simulink model "jumeau_banc_rw"  (R2025b)
settings: Solver=ode23t  StartTime=0.0  StopTime=20  MaxStep=1e-3  RelTol=1e-4
PostLoadFcn:
  | d = fileparts(get_param('jumeau_banc_rw', 'FileName')); addpath(fullfile(d, 'geometrie'), fullfile(d, 'liaison'), fullfile(d, 'pilotage')); clear d
StartFcn:
  | % Jumeau Webots : au lancement, MATLAB envoie les paramètres du Model Workspace à Webots, qui remet le banc en
  | % position de départ, puis ouvre la liaison de télémétrie et la liaison de commande (liaison/pont_banc.m).
  | if strcmp(get_param('jumeau_banc_rw/Procédé', 'LabelModeActiveChoice'), 'Webots')
  |     pont_banc('ouvrir', getVariable(get_param('jumeau_banc_rw', 'ModelWorkspace'), 'config_jumeau'));
  | end
  | pilotage_banc('depart');   % interface de pilotage : nouveau lancement
StopFcn:
  | pont_banc('fermer');
  | pilotage_banc('fin');
model workspace (MATLAB code in the model file):
  | %% Jumeau numérique du banc de stabilisation à 4 roues de réaction (version 3) : paramètres
  | % Ce code est enregistré dans le modèle (Model Explorer > jumeau_banc_rw > Model Workspace).
  | % Origine : (CAO) CAO du banc version 3, (M) mesuré sur le matériel, (F) fiche technique, (Fw) firmware,
  | % (H) hypothèse à mesurer sur le banc. Masses et inerties des pièces : dans chaque bloc de pièce.
  | 
  | %% Montage de l'essai
  | pivot_mm = 25;              % position du pivot de tangage sur le corps : 25, 24, 16, 8, 0, -8 mm (25 : banc équilibré, rangée +24 et paliers remontés de 1 mm)
  | blocage_roulis = 0;         % goupille de blocage : 1 = axe bloqué à 0°, 0 = axe libre
  | blocage_tangage = 0;
  | angle0_roulis_deg = 2;      % position de départ (mise à 0 si l'axe est bloqué)
  | angle0_tangage_deg = -1;
  | g = 9.81;                   % m/s²
  | 
  | %% Pupitre : pilotage manuel des 4 ESC
  | essai_t = 1;                % s, instant de l'échelon d'essai ajouté aux curseurs
  | essai_echelon_us = [0 0 0 0];   % µs, échelon d'essai sur chaque ESC (0 : aucun)
  | 
  | %% Alimentation des ESC
  | V_alim = 12;                % V, alimentation de labo (H : tension réglée)
  | 
  | %% ESC Brushless 30A bidirectionnels (x4)
  | f_trame_esc = 50;           % Hz, une impulsion toutes les 20 ms (Fw : LEDC 50 Hz)
  | imp_neutre = 1500;          % µs, neutre (testé sur le banc)
  | imp_min = 1000;             % µs (Fw)
  | imp_max = 2000;             % µs (Fw)
  | zone_morte_us = 0;          % µs autour du neutre (H)
  | tau_esc = 2e-3;             % s, temps de réponse de l'ESC (H)
  | armement_actif = 1;         % 1 : l'ESC ne pilote le moteur qu'après t_armement au neutre
  | t_armement = 1;             % s (H)
  | fenetre_armement_us = 25;   % µs, écart au neutre accepté pendant l'armement (H)
  | sens_moteurs = [1 1 1 1];   % +1 : au-dessus du neutre, la roue tourne dans le sens +axe (vers l'extérieur) (H : ordre des phases)
  | 
  | %% Moteurs A2212 1400 KV (x4), modèle équivalent continu
  | KV = 1400;                  % tr/min/V (F)
  | Ke = 60/(2*pi*KV);          % V.s/rad
  | Kt = Ke;                    % N.m/A
  | R_moteur = 0.08;            % ohm (H)
  | L_moteur = 30e-6;           % H (H)
  | f_roue = 5e-6;              % N.m.s/rad, frottement visqueux des roulements du moteur (H)
  | 
  | %% Cardan
  | butee_deg = 20;             % débattement de chaque axe (CAO)
  | k_butee = 20;               % N.m/rad, contact goupille-lumière (H)
  | c_butee = 0.2;              % N.m.s/rad (H)
  | b_cardan = 1e-4;            % N.m.s/rad, frottement des roulements 625 (H)
  | k_cables = 0;               % N.m/rad, raideur des deux câbles vers la table (H)
  | 
  | %% BNO055 (mode fusion)
  | T_bno = 0.01;               % s, données de fusion à 100 Hz (F)
  | bruit_bno = 1;              % 1 : bruit de mesure, 0 : capteur parfait
  | sigma_angle_deg = 0.05;     % ° (H)
  | sigma_gyro_dps = 0.1;       % °/s (H)
  | sigma_acc = 0.02;           % m/s² (H)
  | R_montage_bno = eye(3);     % axes du capteur dans le repère du dispositif : eye(3) = remappage AXIS_MAP réglé
  |                             % (la carte est tournée de 90° dans la CAO)
  | 
  | %% Capteurs de vitesse TCRT5000 (x4) : un front à chaque rayon du disque
  | n_rayons = 4;               % rayons du disque vus par tour (CAO : disque d'origine)
  | T_tcrt = 1e-3;              % s, pas de calcul du capteur (les fronts sont datés par interpolation, comme un chronomètre en µs)
  | t_arret_tcrt = 0.2;         % s sans front : la vitesse mesurée retombe à 0 (Fw, à fixer)
  | 
  | %% Pont vers le jumeau Webots (et, plus tard, vers l'ESP32 du banc réel)
  | T_pont = 0.01;              % s, une trame de commande et une trame de télémétrie toutes les 10 ms
  | 
  | %% Essai : maintien au départ et perturbation
  | t_lacher = 2;                % s, le dispositif est tenu à la main à sa position de départ jusqu'à cet instant (0 : libre dès le départ)
  | k_main = 5;                  % N.m/rad, raideur de la main qui tient le dispositif
  | c_main = 0.3;                % N.m.s/rad, son amortissement
  | perturbation_t = 7;          % s, instant de la poussée d'essai
  | perturbation_duree = 0.2;    % s
  | perturbation_couple = [0.02 0.02];   % N.m, couple de la poussée sur [roulis tangage], programmée (0 : aucune ; l'interface de pilotage en ajoute)
  | 
  | %% Grandeurs dérivées
  | assert(any(pivot_mm == [25 24 16 8 0 -8]), 'pivot_mm : 25, 24, 16, 8, 0, -8');
  | q0_deg = [angle0_roulis_deg angle0_tangage_deg] .* ([blocage_roulis blocage_tangage] == 0);
  | config_jumeau = [pivot_mm; blocage_roulis; blocage_tangage; q0_deg(:); V_alim; f_trame_esc; imp_neutre; imp_min; imp_max; ...
  |     zone_morte_us; tau_esc; armement_actif; t_armement; fenetre_armement_us; sens_moteurs(:); Ke; Kt; R_moteur; L_moteur; ...
  |     f_roue; butee_deg; k_butee; c_butee; b_cardan; k_cables; g; T_bno; bruit_bno; sigma_angle_deg; sigma_gyro_dps; ...
  |     sigma_acc; n_rayons; t_arret_tcrt; T_tcrt; R_montage_bno(:); T_pont; t_lacher; k_main; c_main];   % 51 valeurs envoyées au jumeau Webots au lancement
  | 
  | %% Commande bas niveau : une boucle de vitesse par roue, avec observateur CFO (méthode du TP2, ramenée à la vitesse)
  | J_roue = 1.562e-4;          % kg.m², inertie d'une roue autour de son axe : disque, vis, cloche du moteur (CAO)
  | T_cbn = 1/f_trame_esc;      % s, période de calcul de la commande : celle des ESC, qui ne lisent qu'une impulsion toutes les 20 ms
  | wc_roue = [10 10 10 10];    % rad/s, rapidité du suivi de vitesse de chaque roue (pôle de l'erreur en -wc)
  | wo_roue = [5 5 5 5];        % rad/s, rapidité du CFO de chaque roue (pôles en -wo et -4 wo) ; au-delà de 10, il devient instable à 20 ms
  | imp_cmd_min = 1375;         % µs, limites des impulsions commandées : vitesse conseillée des disques, 3 900 tr/min
  | imp_cmd_max = 1625;         % µs
  | w_aveugle = 45;             % rad/s, en dessous (vitesse du modèle), le TCRT5000 voit mal la roue : le CFO ne se corrige plus sur la mesure
  | 
  | %% Consigne d'essai des roues : ajoutée à la consigne qui vient de la conversion (0 tant qu'elle est vide)
  | essai_roue_t1 = 2;                  % s, départ vers le premier palier
  | essai_roue_vitesse1 = [0 0 0 0];  % rad/s, premier palier de chaque roue (0 : la roue reste à l'arrêt)
  | essai_roue_t2 = 6;                  % s, départ vers le second palier
  | essai_roue_vitesse2 = [0 0 0 0];    % rad/s, second palier de chaque roue
  | essai_roue_acc = 300;               % rad/s², pente des rampes entre les paliers
  | 
  | %% Commande bas niveau : grandeurs calculées
  | % modèle local d'une roue : d(omega)/dt = -a1 omega + a0 V + d
  | a0_roue = Kt/(R_moteur*J_roue) * [1 1 1 1];                % rad/s² par volt
  | a1_roue = (Kt*Ke/R_moteur + f_roue)/J_roue * [1 1 1 1];    % 1/s
  | K_roue = wc_roue - a1_roue;                                % retour d'état : erreur en -(a1 + K) = -wc
  | l1_roue = 5*wo_roue;                                       % CFO
  | lambda_roue = 4/5*wo_roue;
  | 
  | %% Référence : angles demandés au dispositif, en polynômes de degré 5 entre deux paliers
  | ref_t = [2 12];              % s, instant de départ vers chaque palier
  | ref_roulis_deg = [0 5];      % °, roulis demandé à chaque palier
  | ref_tangage_deg = [0 0];     % °, tangage demandé à chaque palier
  | ref_duree = 1.5;             % s, durée du passage d'un palier au suivant
  | 
  | %% Commande haut niveau : une boucle par axe [roulis tangage], placement de pôles basé sur l'observateur CFO (TP2)
  | T_chn = T_cbn;               % s, période de calcul : celle de la commande bas niveau et des ESC
  | t_depart = t_lacher;         % s, mise en marche de la commande : au moment où la main lâche le dispositif
  | wc_axe = [4 4];              % rad/s, rapidité du suivi d'angle de chaque axe
  | xi_axe = [1 1];              % amortissement
  | wo_axe = [3 3];              % rad/s, rapidité du CFO de chaque axe (pôles en -wo et -4 wo, double) ; au-delà de 4, le couple s'agite
  | desat_active = 0;            % 1 : la référence est décalée pour ramener les roues vers leur vitesse de repos
  | T_desat = 5;                 % s, constante de temps de ce retour
  | desat_max_deg = 15;          % °, décalage maximal de la référence
  | 
  | %% Conversion : couples des deux axes vers les 4 roues
  | w_repos = 200;               % rad/s, vitesse de repos des 4 roues : elles tournent toujours, le TCRT5000 les voit toujours
  | t_roues = t_armement + 0.2;  % s, mise en rotation des roues, une fois les ESC armés
  | acc_roue_max = 300;          % rad/s², accélération maximale demandée à une roue
  | w_roue_min = 60;             % rad/s, vitesses limites demandées à une roue
  | w_roue_max = 400;            % rad/s (disques : 3 900 tr/min conseillés, soit 408 rad/s)
  | 
  | %% Masses et inerties utilisées par la commande (CAO du banc version 3)
  | m_disp = 1.2615;             % kg, dispositif et ses 4 roues
  | zG_disp = 24.977e-3;         % m, hauteur de son centre de masse sur le corps (le pivot est à pivot_mm)
  | Ixx_disp_24 = 8.2684e-3;     % kg.m², inertie du dispositif autour du roulis, pivot à +24 mm
  | Iyy_disp_24 = 8.2786e-3;     % kg.m², autour du tangage, pivot à +24 mm
  | m_croix = 0.0755;            % kg, croisillon et paliers (ne tournent qu'en roulis)
  | zG_croix = 0.257e-3;         % m, hauteur de leur centre de masse au-dessus de l'axe de roulis
  | Ixx_croix = 2.073e-4;        % kg.m²
  | 
  | %% Commande haut niveau et conversion : grandeurs calculées
  | % modèle local d'un axe : d²(theta)/dt² = -a1 d(theta)/dt + a0 C + d, avec C le couple demandé aux roues
  | hz = zG_disp - pivot_mm/1000;                                    % m, centre de masse du dispositif au-dessus du pivot
  | I_axe = [Ixx_disp_24 + Ixx_croix, Iyy_disp_24] + m_disp*(hz^2 - (zG_disp - 0.024)^2) - 2*J_roue;   % kg.m²
  | mgh_axe = g*[m_disp*hz + m_croix*zG_croix, m_disp*hz];           % N.m/rad, couple de pesanteur par radian d'inclinaison
  | a0_axe = 1./I_axe;                                               % rad/s² par N.m
  | a1_axe = b_cardan./I_axe;                                        % 1/s
  | k1_axe = wc_axe.^2;                                              % retour d'état : s² + 2 xi wc s + wc²
  | k2_axe = 2*xi_axe.*wc_axe - a1_axe;
  | l1_axe = 9*wo_axe;                                               % CFO du TP2
  | l2_axe = 12*wo_axe.^2;
  | lambda_axe = 4/3*wo_axe;
  | C_max = 2*J_roue*cosd(45)*acc_roue_max;                          % N.m, couple maximal demandé sur un axe
  | k_desat = desat_active.*sign(mgh_axe + (mgh_axe == 0))./(max(abs(mgh_axe), 1e-3)*T_desat);            % rad par N.m.s
  | sx_roues = [1 -1 -1 1];                                          % signe de cos(45°, 135°, 225°, 315°) : part de chaque roue sur le roulis
  | sy_roues = [1 1 -1 -1];                                          % signe de sin : part sur le tangage
  | M_conv = -[sx_roues(:) sy_roues(:)]/(4*J_roue*cosd(45));         % accélération des 4 roues pour un couple [roulis; tangage]
  | 
  | %% Perception : des mesures à l'état du banc
  | T_perception = T_bno;        % s, période de calcul : celle du BNO055
  | tau_desequilibre = 2;        % s, constante de temps du filtre du couple extérieur et du déséquilibre
  | 
  | %% Pilotage par l'interface (pilotage/pilote_banc.m)
  | manche_max_deg = 15;         % °, limite de sécurité de l'inclinaison demandée par le manche (l'interface règle l'amplitude)
  | w_manche = 3;                % rad/s, rapidité avec laquelle la référence rejoint le manche (second ordre critique)
  | T_affichage = 0.1;           % s, rafraîchissement de l'interface
undefined symbols (not defined in the file): DiscIntNeverNeededParam, X, Y, Z
libraries: sm_lib x256, nesl_utility x24, simulink x7
(part 3 of 8)

== system jumeau_banc_rw/Procédé/Jumeau Simscape/Mécanique (CAO version 3)/Croisillon (tourne en roulis) ==
  Collier 1 : sm_lib/Body Elements/File Solid  Description=|  ExtGeomFileName=RW-05_Collier.stl  UnitType=Custom  ExtGeomFileUnits=mm  StepReaderType=HEX  ExportConvexHullGeometry=off  InertiaType=Custom  BasedOnType=DensityFromFile  Density=1000  DensityUnits=kg/m^3  Mass=0.005537042  MassUnits=kg  CenterOfMass=[-0.00035108193 2.2209262e-05 0.0029842808]  CenterOfMassUnits=m  MomentsOfInertia=[3.8543243e-07 3.7829745e-07 7.2925271e-07]  MomentsOfInertiaUnits=kg*m^2  ProductsOfInertia=[-1.9330542e-12 3.0559842e-11 -4.3174034e-11]  ProductsOfInertiaUnits=kg*m^2  GraphicType=FromGeometry  MarkerShape=Sphere  MarkerSize=10  GraphicVisPropType=SimpleVisualProperties  GraphicDiffuseColor=[0.867 0.518 0.322]  GraphicOpacity=1  GraphicSpecularColor=[0.5 0.5 0.5 1.0]  GraphicAmbientColor=[0.15 0.15 0.15 1.0]  GraphicEmissiveColor=[0.0 0.0 0.0 1.0]  GraphicShininess=75  DoExposeReferenceFrame=on  SerializedFrames=<Frames/>
      | Pièce CAO : Collier 1 (RW-05_Collier)
      | Masse 5.54 g : PLA plein (hypothèse de conception), 1240 kg/m³.
      | Centre de masse et inertie : calculés sur la géométrie de la CAO.
  Collier 2 : sm_lib/Body Elements/File Solid  Description=|  ExtGeomFileName=RW-05_Collier.stl  UnitType=Custom  ExtGeomFileUnits=mm  StepReaderType=HEX  ExportConvexHullGeometry=off  InertiaType=Custom  BasedOnType=DensityFromFile  Density=1000  DensityUnits=kg/m^3  Mass=0.005537042  MassUnits=kg  CenterOfMass=[-0.00035108193 2.2209262e-05 0.0029842808]  CenterOfMassUnits=m  MomentsOfInertia=[3.8543243e-07 3.7829745e-07 7.2925271e-07]  MomentsOfInertiaUnits=kg*m^2  ProductsOfInertia=[-1.9330542e-12 3.0559842e-11 -4.3174034e-11]  ProductsOfInertiaUnits=kg*m^2  GraphicType=FromGeometry  MarkerShape=Sphere  MarkerSize=10  GraphicVisPropType=SimpleVisualProperties  GraphicDiffuseColor=[0.867 0.518 0.322]  GraphicOpacity=1  GraphicSpecularColor=[0.5 0.5 0.5 1.0]  GraphicAmbientColor=[0.15 0.15 0.15 1.0]  GraphicEmissiveColor=[0.0 0.0 0.0 1.0]  GraphicShininess=75  DoExposeReferenceFrame=on  SerializedFrames=<Frames/>
      | Pièce CAO : Collier 2 (RW-05_Collier)
      | Masse 5.54 g : PLA plein (hypothèse de conception), 1240 kg/m³.
      | Centre de masse et inertie : calculés sur la géométrie de la CAO.
  Croisillon : sm_lib/Body Elements/File Solid  Description=|  ExtGeomFileName=RW-06_Croisillon.stl  UnitType=Custom  ExtGeomFileUnits=mm  StepReaderType=HEX  ExportConvexHullGeometry=off  InertiaType=Custom  BasedOnType=DensityFromFile  Density=1000  DensityUnits=kg/m^3  Mass=0.025623078  MassUnits=kg  CenterOfMass=[-4.3032906e-14 1.5829923e-12 -4.8306735e-05]  CenterOfMassUnits=m  MomentsOfInertia=[3.4638965e-06 3.4316654e-06 3.4293676e-06]  MomentsOfInertiaUnits=kg*m^2  ProductsOfInertia=[-6.2250551e-17 3.045946e-18 -4.6836641e-17]  ProductsOfInertiaUnits=kg*m^2  GraphicType=FromGeometry  MarkerShape=Sphere  MarkerSize=10  GraphicVisPropType=SimpleVisualProperties  GraphicDiffuseColor=[0.91 0.639 0.239]  GraphicOpacity=1  GraphicSpecularColor=[0.5 0.5 0.5 1.0]  GraphicAmbientColor=[0.15 0.15 0.15 1.0]  GraphicEmissiveColor=[0.0 0.0 0.0 1.0]  GraphicShininess=75  DoExposeReferenceFrame=on  SerializedFrames=<Frames/>
      | Pièce CAO : Croisillon (RW-06_Croisillon)
      | Masse 25.62 g : PLA plein (hypothèse de conception), 1240 kg/m³.
      | Centre de masse et inertie : calculés sur la géométrie de la CAO.
  Entretoise de roulis 1 : sm_lib/Body Elements/File Solid  Description=|  ExtGeomFileName=RW-23_Entretoise-roulis-8x4.stl  UnitType=Custom  ExtGeomFileUnits=mm  StepReaderType=HEX  ExportConvexHullGeometry=off  InertiaType=Custom  BasedOnType=DensityFromFile  Density=1000  DensityUnits=kg/m^3  Mass=9.5479284e-05  MassUnits=kg  CenterOfMass=[-2.0837187e-19 -2.3504414e-20 0.002]  CenterOfMassUnits=m  MomentsOfInertia=[6.6443636e-10 6.6443636e-10 1.0742613e-09]  MomentsOfInertiaUnits=kg*m^2  ProductsOfInertia=[4.6214258e-28 1.1368684e-26 -3.8597625e-27]  ProductsOfInertiaUnits=kg*m^2  GraphicType=FromGeometry  MarkerShape=Sphere  MarkerSize=10  GraphicVisPropType=SimpleVisualProperties  GraphicDiffuseColor=[0.867 0.518 0.322]  GraphicOpacity=1  GraphicSpecularColor=[0.5 0.5 0.5 1.0]  GraphicAmbientColor=[0.15 0.15 0.15 1.0]  GraphicEmissiveColor=[0.0 0.0 0.0 1.0]  GraphicShininess=75  DoExposeReferenceFrame=on  SerializedFrames=<Frames/>
      | Pièce CAO : Entretoise de roulis 1 (RW-23_Entretoise-roulis-8x4)
      | Masse 0.10 g : PLA imprimé, 2 parois et 15 % de remplissage (hypothèse de conception), 800 kg/m³.
      | Centre de masse et inertie : calculés sur la géométrie de la CAO.
  Entretoise de roulis 2 : sm_lib/Body Elements/File Solid  Description=|  ExtGeomFileName=RW-23_Entretoise-roulis-8x4.stl  UnitType=Custom  ExtGeomFileUnits=mm  StepReaderType=HEX  ExportConvexHullGeometry=off  InertiaType=Custom  BasedOnType=DensityFromFile  Density=1000  DensityUnits=kg/m^3  Mass=9.5479284e-05  MassUnits=kg  CenterOfMass=[-2.0837187e-19 -2.3504414e-20 0.002]  CenterOfMassUnits=m  MomentsOfInertia=[6.6443636e-10 6.6443636e-10 1.0742613e-09]  MomentsOfInertiaUnits=kg*m^2  ProductsOfInertia=[4.6214258e-28 1.1368684e-26 -3.8597625e-27]  ProductsOfInertiaUnits=kg*m^2  GraphicType=FromGeometry  MarkerShape=Sphere  MarkerSize=10  GraphicVisPropType=SimpleVisualProperties  GraphicDiffuseColor=[0.867 0.518 0.322]  GraphicOpacity=1  GraphicSpecularColor=[0.5 0.5 0.5 1.0]  GraphicAmbientColor=[0.15 0.15 0.15 1.0]  GraphicEmissiveColor=[0.0 0.0 0.0 1.0]  GraphicShininess=75  DoExposeReferenceFrame=on  SerializedFrames=<Frames/>
      | Pièce CAO : Entretoise de roulis 2 (RW-23_Entretoise-roulis-8x4)
      | Masse 0.10 g : PLA imprimé, 2 parois et 15 % de remplissage (hypothèse de conception), 800 kg/m³.
      | Centre de masse et inertie : calculés sur la géométrie de la CAO.
  Goupille de butée de roulis : sm_lib/Body Elements/File Solid  Description=|  ExtGeomFileName=RW-24_Goupille-3x16.stl  UnitType=Custom  ExtGeomFileUnits=mm  StepReaderType=HEX  ExportConvexHullGeometry=off  InertiaType=Custom  BasedOnType=DensityFromFile  Density=1000  DensityUnits=kg/m^3  Mass=0.00088781408  MassUnits=kg  CenterOfMass=[-3.8480785e-19 5.0963439e-20 0.008]  CenterOfMassUnits=m  MomentsOfInertia=[1.9439429e-08 1.9439429e-08 9.9879084e-10]  MomentsOfInertiaUnits=kg*m^2  ProductsOfInertia=[2.3957297e-27 -4.1833204e-25 1.4074912e-26]  ProductsOfInertiaUnits=kg*m^2  GraphicType=FromGeometry  MarkerShape=Sphere  MarkerSize=10  GraphicVisPropType=SimpleVisualProperties  GraphicDiffuseColor=[0.314 0.314 0.314]  GraphicOpacity=1  GraphicSpecularColor=[0.5 0.5 0.5 1.0]  GraphicAmbientColor=[0.15 0.15 0.15 1.0]  GraphicEmissiveColor=[0.0 0.0 0.0 1.0]  GraphicShininess=75  DoExposeReferenceFrame=on  SerializedFrames=<Frames/>
      | Pièce CAO : Goupille de butée de roulis (RW-24_Goupille-3x16)
      | Masse 0.89 g : acier, 7850 kg/m³.
      | Centre de masse et inertie : calculés sur la géométrie de la CAO.
  Goupille de butée de tangage : sm_lib/Body Elements/File Solid  Description=|  ExtGeomFileName=RW-24_Goupille-3x16.stl  UnitType=Custom  ExtGeomFileUnits=mm  StepReaderType=HEX  ExportConvexHullGeometry=off  InertiaType=Custom  BasedOnType=DensityFromFile  Density=1000  DensityUnits=kg/m^3  Mass=0.00088781408  MassUnits=kg  CenterOfMass=[-3.8480785e-19 5.0963439e-20 0.008]  CenterOfMassUnits=m  MomentsOfInertia=[1.9439429e-08 1.9439429e-08 9.9879084e-10]  MomentsOfInertiaUnits=kg*m^2  ProductsOfInertia=[2.3957297e-27 -4.1833204e-25 1.4074912e-26]  ProductsOfInertiaUnits=kg*m^2  GraphicType=FromGeometry  MarkerShape=Sphere  MarkerSize=10  GraphicVisPropType=SimpleVisualProperties  GraphicDiffuseColor=[0.314 0.314 0.314]  GraphicOpacity=1  GraphicSpecularColor=[0.5 0.5 0.5 1.0]  GraphicAmbientColor=[0.15 0.15 0.15 1.0]  GraphicEmissiveColor=[0.0 0.0 0.0 1.0]  GraphicShininess=75  DoExposeReferenceFrame=on  SerializedFrames=<Frames/>
      | Pièce CAO : Goupille de butée de tangage (RW-24_Goupille-3x16)
      | Masse 0.89 g : acier, 7850 kg/m³.
      | Centre de masse et inertie : calculés sur la géométrie de la CAO.
  Pose Collier 1 : sm_lib/Frames and Transforms/Rigid Transform  RotationMethod=RotationMatrix  FollAlignAxisA=+X  BaseAlignAxisA=+Y  FollAlignAxisB=+Y  BaseAlignAxisB=+Z  RotationStandardAxis=+Z  RotationAngle=0  RotationAngleUnits=deg  RotationArbitraryAxis=[0 0 1]  RotationSequenceAxes=FollowerAxes  RotationSequence=XYX  RotationSequenceAngles=[0 0 0]  RotationSequenceAnglesUnits=deg  RotationMatrix=[-1 0 0;0 0 1;0 1 0]  Quaternion=[1 0 0 0]  TranslationMethod=Cartesian  TranslationCartesianOffset=[0 88.5 0]  TranslationCartesianOffsetUnits=mm  TranslationStandardAxis=+Z  TranslationStandardOffset=0  TranslationStandardOffsetUnits=m  TranslationROffset=0  TranslationROffsetUnits=m  TranslationThetaOffset=0  TranslationThetaOffsetUnits=deg  TranslationZOffset=0  TranslationZOffsetUnits=m
  Pose Collier 2 : sm_lib/Frames and Transforms/Rigid Transform  RotationMethod=RotationMatrix  FollAlignAxisA=+X  BaseAlignAxisA=+Y  FollAlignAxisB=+Y  BaseAlignAxisB=+Z  RotationStandardAxis=+Z  RotationAngle=0  RotationAngleUnits=deg  RotationArbitraryAxis=[0 0 1]  RotationSequenceAxes=FollowerAxes  RotationSequence=XYX  RotationSequenceAngles=[0 0 0]  RotationSequenceAnglesUnits=deg  RotationMatrix=[1 0 0;0 0 -1;0 1 0]  Quaternion=[1 0 0 0]  TranslationMethod=Cartesian  TranslationCartesianOffset=[0 -88.5 0]  TranslationCartesianOffsetUnits=mm  TranslationStandardAxis=+Z  TranslationStandardOffset=0  TranslationStandardOffsetUnits=m  TranslationROffset=0  TranslationROffsetUnits=m  TranslationThetaOffset=0  TranslationThetaOffsetUnits=deg  TranslationZOffset=0  TranslationZOffsetUnits=m
  Pose Entretoise de roulis 1 : sm_lib/Frames and Transforms/Rigid Transform  RotationMethod=RotationMatrix  FollAlignAxisA=+X  BaseAlignAxisA=+Y  FollAlignAxisB=+Y  BaseAlignAxisB=+Z  RotationStandardAxis=+Z  RotationAngle=0  RotationAngleUnits=deg  RotationArbitraryAxis=[0 0 1]  RotationSequenceAxes=FollowerAxes  RotationSequence=XYX  RotationSequenceAngles=[0 0 0]  RotationSequenceAnglesUnits=deg  RotationMatrix=[0 0 1;1 0 0;0 1 0]  Quaternion=[1 0 0 0]  TranslationMethod=Cartesian  TranslationCartesianOffset=[14 0 0]  TranslationCartesianOffsetUnits=mm  TranslationStandardAxis=+Z  TranslationStandardOffset=0  TranslationStandardOffsetUnits=m  TranslationROffset=0  TranslationROffsetUnits=m  TranslationThetaOffset=0  TranslationThetaOffsetUnits=deg  TranslationZOffset=0  TranslationZOffsetUnits=m
  Pose Entretoise de roulis 2 : sm_lib/Frames and Transforms/Rigid Transform  RotationMethod=RotationMatrix  FollAlignAxisA=+X  BaseAlignAxisA=+Y  FollAlignAxisB=+Y  BaseAlignAxisB=+Z  RotationStandardAxis=+Z  RotationAngle=0  RotationAngleUnits=deg  RotationArbitraryAxis=[0 0 1]  RotationSequenceAxes=FollowerAxes  RotationSequence=XYX  RotationSequenceAngles=[0 0 0]  RotationSequenceAnglesUnits=deg  RotationMatrix=[0 0 -1;1 0 0;0 -1 0]  Quaternion=[1 0 0 0]  TranslationMethod=Cartesian  TranslationCartesianOffset=[-14 0 0]  TranslationCartesianOffsetUnits=mm  TranslationStandardAxis=+Z  TranslationStandardOffset=0  TranslationStandardOffsetUnits=m  TranslationROffset=0  TranslationROffsetUnits=m  TranslationThetaOffset=0  TranslationThetaOffsetUnits=deg  TranslationZOffset=0  TranslationZOffsetUnits=m
  Pose Goupille de butée de roulis : sm_lib/Frames and Transforms/Rigid Transform  RotationMethod=RotationMatrix  FollAlignAxisA=+X  BaseAlignAxisA=+Y  FollAlignAxisB=+Y  BaseAlignAxisB=+Z  RotationStandardAxis=+Z  RotationAngle=0  RotationAngleUnits=deg  RotationArbitraryAxis=[0 0 1]  RotationSequenceAxes=FollowerAxes  RotationSequence=XYX  RotationSequenceAngles=[0 0 0]  RotationSequenceAnglesUnits=deg  RotationMatrix=[0 0 1;1 0 0;0 1 0]  Quaternion=[1 0 0 0]  TranslationMethod=Cartesian  TranslationCartesianOffset=[8 0 11.5]  TranslationCartesianOffsetUnits=mm  TranslationStandardAxis=+Z  TranslationStandardOffset=0  TranslationStandardOffsetUnits=m  TranslationROffset=0  TranslationROffsetUnits=m  TranslationThetaOffset=0  TranslationThetaOffsetUnits=deg  TranslationZOffset=0  TranslationZOffsetUnits=m
  Pose Goupille de butée de tangage : sm_lib/Frames and Transforms/Rigid Transform  RotationMethod=RotationMatrix  FollAlignAxisA=+X  BaseAlignAxisA=+Y  FollAlignAxisB=+Y  BaseAlignAxisB=+Z  RotationStandardAxis=+Z  RotationAngle=0  RotationAngleUnits=deg  RotationArbitraryAxis=[0 0 1]  RotationSequenceAxes=FollowerAxes  RotationSequence=XYX  RotationSequenceAngles=[0 0 0]  RotationSequenceAnglesUnits=deg  RotationMatrix=[1 0 0;0 0 1;0 -1 0]  Quaternion=[1 0 0 0]  TranslationMethod=Cartesian  TranslationCartesianOffset=[0 82.5 11.5]  TranslationCartesianOffsetUnits=mm  TranslationStandardAxis=+Z  TranslationStandardOffset=0  TranslationStandardOffsetUnits=m  TranslationROffset=0  TranslationROffsetUnits=m  TranslationThetaOffset=0  TranslationThetaOffsetUnits=deg  TranslationZOffset=0  TranslationZOffsetUnits=m
  Pose Tige de tangage : sm_lib/Frames and Transforms/Rigid Transform  RotationMethod=RotationMatrix  FollAlignAxisA=+X  BaseAlignAxisA=+Y  FollAlignAxisB=+Y  BaseAlignAxisB=+Z  RotationStandardAxis=+Z  RotationAngle=0  RotationAngleUnits=deg  RotationArbitraryAxis=[0 0 1]  RotationSequenceAxes=FollowerAxes  RotationSequence=XYX  RotationSequenceAngles=[0 0 0]  RotationSequenceAnglesUnits=deg  RotationMatrix=[1 0 0;0 0 1;0 -1 0]  Quaternion=[1 0 0 0]  TranslationMethod=Cartesian  TranslationCartesianOffset=[0 0 0]  TranslationCartesianOffsetUnits=mm  TranslationStandardAxis=+Z  TranslationStandardOffset=0  TranslationStandardOffsetUnits=m  TranslationROffset=0  TranslationROffsetUnits=m  TranslationThetaOffset=0  TranslationThetaOffsetUnits=deg  TranslationZOffset=0  TranslationZOffsetUnits=m
  Pose Vis épaulée 1 : sm_lib/Frames and Transforms/Rigid Transform  RotationMethod=RotationMatrix  FollAlignAxisA=+X  BaseAlignAxisA=+Y  FollAlignAxisB=+Y  BaseAlignAxisB=+Z  RotationStandardAxis=+Z  RotationAngle=0  RotationAngleUnits=deg  RotationArbitraryAxis=[0 0 1]  RotationSequenceAxes=FollowerAxes  RotationSequence=XYX  RotationSequenceAngles=[0 0 0]  RotationSequenceAnglesUnits=deg  RotationMatrix=[0 0 -1;1 0 0;0 -1 0]  Quaternion=[1 0 0 0]  TranslationMethod=Cartesian  TranslationCartesianOffset=[23 0 0]  TranslationCartesianOffsetUnits=mm  TranslationStandardAxis=+Z  TranslationStandardOffset=0  TranslationStandardOffsetUnits=m  TranslationROffset=0  TranslationROffsetUnits=m  TranslationThetaOffset=0  TranslationThetaOffsetUnits=deg  TranslationZOffset=0  TranslationZOffsetUnits=m
  Pose Vis épaulée 2 : sm_lib/Frames and Transforms/Rigid Transform  RotationMethod=RotationMatrix  FollAlignAxisA=+X  BaseAlignAxisA=+Y  FollAlignAxisB=+Y  BaseAlignAxisB=+Z  RotationStandardAxis=+Z  RotationAngle=0  RotationAngleUnits=deg  RotationArbitraryAxis=[0 0 1]  RotationSequenceAxes=FollowerAxes  RotationSequence=XYX  RotationSequenceAngles=[0 0 0]  RotationSequenceAnglesUnits=deg  RotationMatrix=[0 0 1;1 0 0;0 1 0]  Quaternion=[1 0 0 0]  TranslationMethod=Cartesian  TranslationCartesianOffset=[-23 0 0]  TranslationCartesianOffsetUnits=mm  TranslationStandardAxis=+Z  TranslationStandardOffset=0  TranslationStandardOffsetUnits=m  TranslationROffset=0  TranslationROffsetUnits=m  TranslationThetaOffset=0  TranslationThetaOffsetUnits=deg  TranslationZOffset=0  TranslationZOffsetUnits=m
  Tige de tangage : sm_lib/Body Elements/File Solid  Description=|  ExtGeomFileName=RW-21_Tige-5x200.stl  UnitType=Custom  ExtGeomFileUnits=mm  StepReaderType=HEX  ExportConvexHullGeometry=off  InertiaType=Custom  BasedOnType=DensityFromFile  Density=1000  DensityUnits=kg/m^3  Mass=0.030826878  MassUnits=kg  CenterOfMass=[3.4740139e-19 -9.3482873e-20 0]  CenterOfMassUnits=m  MomentsOfInertia=[0.00010280443 0.00010280443 9.6333993e-08]  MomentsOfInertiaUnits=kg*m^2  ProductsOfInertia=[-8.2139303e-24 -1.1423253e-22 1.106194e-23]  ProductsOfInertiaUnits=kg*m^2  GraphicType=FromGeometry  MarkerShape=Sphere  MarkerSize=10  GraphicVisPropType=SimpleVisualProperties  GraphicDiffuseColor=[0.2 0.2 0.2]  GraphicOpacity=1  GraphicSpecularColor=[0.5 0.5 0.5 1.0]  GraphicAmbientColor=[0.15 0.15 0.15 1.0]  GraphicEmissiveColor=[0.0 0.0 0.0 1.0]  GraphicShininess=75  DoExposeReferenceFrame=on  SerializedFrames=<Frames/>
      | Pièce CAO : Tige de tangage (RW-21_Tige-5x200)
      | Masse 30.83 g : acier, 7850 kg/m³.
      | Centre de masse et inertie : calculés sur la géométrie de la CAO.
  Vis épaulée 1 : sm_lib/Body Elements/File Solid  Description=|  ExtGeomFileName=RW-22_Vis-epaulee-5x10-M4.stl  UnitType=Custom  ExtGeomFileUnits=mm  StepReaderType=HEX  ExportConvexHullGeometry=off  InertiaType=Custom  BasedOnType=DensityFromFile  Density=1000  DensityUnits=kg/m^3  Mass=0.003  MassUnits=kg  CenterOfMass=[-4.1357308e-19 -6.3568799e-20 0.0032357143]  CenterOfMassUnits=m  MomentsOfInertia=[1.0565385e-07 1.0565385e-07 1.7426786e-08]  MomentsOfInertiaUnits=kg*m^2  ProductsOfInertia=[-6.72648e-25 -5.787069e-24 1.5426199e-24]  ProductsOfInertiaUnits=kg*m^2  GraphicType=FromGeometry  MarkerShape=Sphere  MarkerSize=10  GraphicVisPropType=SimpleVisualProperties  GraphicDiffuseColor=[0.533 0.533 0.533]  GraphicOpacity=1  GraphicSpecularColor=[0.5 0.5 0.5 1.0]  GraphicAmbientColor=[0.15 0.15 0.15 1.0]  GraphicEmissiveColor=[0.0 0.0 0.0 1.0]  GraphicShininess=75  DoExposeReferenceFrame=on  SerializedFrames=<Frames/>
      | Pièce CAO : Vis épaulée 1 (RW-22_Vis-epaulee-5x10-M4)
      | Masse 3.00 g : vis épaulée ISO 7379, catalogue, 3 g répartis sur le volume de la CAO.
      | Centre de masse et inertie : calculés sur la géométrie de la CAO.
  Vis épaulée 2 : sm_lib/Body Elements/File Solid  Description=|  ExtGeomFileName=RW-22_Vis-epaulee-5x10-M4.stl  UnitType=Custom  ExtGeomFileUnits=mm  StepReaderType=HEX  ExportConvexHullGeometry=off  InertiaType=Custom  BasedOnType=DensityFromFile  Density=1000  DensityUnits=kg/m^3  Mass=0.003  MassUnits=kg  CenterOfMass=[-4.1357308e-19 -6.3568799e-20 0.0032357143]  CenterOfMassUnits=m  MomentsOfInertia=[1.0565385e-07 1.0565385e-07 1.7426786e-08]  MomentsOfInertiaUnits=kg*m^2  ProductsOfInertia=[-6.72648e-25 -5.787069e-24 1.5426199e-24]  ProductsOfInertiaUnits=kg*m^2  GraphicType=FromGeometry  MarkerShape=Sphere  MarkerSize=10  GraphicVisPropType=SimpleVisualProperties  GraphicDiffuseColor=[0.533 0.533 0.533]  GraphicOpacity=1  GraphicSpecularColor=[0.5 0.5 0.5 1.0]  GraphicAmbientColor=[0.15 0.15 0.15 1.0]  GraphicEmissiveColor=[0.0 0.0 0.0 1.0]  GraphicShininess=75  DoExposeReferenceFrame=on  SerializedFrames=<Frames/>
      | Pièce CAO : Vis épaulée 2 (RW-22_Vis-epaulee-5x10-M4)
      | Masse 3.00 g : vis épaulée ISO 7379, catalogue, 3 g répartis sur le volume de la CAO.
      | Centre de masse et inertie : calculés sur la géométrie de la CAO.
  F : PMIOPort  Side=Left
  connections:
  Croisillon/RConn1 -- F/RConn1 -- Pose Tige de tangage/LConn1 -- Pose Entretoise de roulis 1/LConn1 -- Pose Vis épaulée 1/LConn1 -- Pose Collier 1/LConn1 -- Pose Entretoise de roulis 2/LConn1 -- Pose Vis épaulée 2/LConn1 -- Pose Collier 2/LConn1 -- Pose Goupille de butée de roulis/LConn1 -- Pose Goupille de butée de tangage/LConn1
  Pose Tige de tangage/RConn1 -- Tige de tangage/RConn1
  Pose Entretoise de roulis 1/RConn1 -- Entretoise de roulis 1/RConn1
  Pose Vis épaulée 1/RConn1 -- Vis épaulée 1/RConn1
  Pose Collier 1/RConn1 -- Collier 1/RConn1
  Pose Entretoise de roulis 2/RConn1 -- Entretoise de roulis 2/RConn1
  Pose Vis épaulée 2/RConn1 -- Vis épaulée 2/RConn1
  Pose Collier 2/RConn1 -- Collier 2/RConn1
  Pose Goupille de butée de roulis/RConn1 -- Goupille de butée de roulis/RConn1
  Pose Goupille de butée de tangage/RConn1 -- Goupille de butée de tangage/RConn1
